simulink model "updated_simulation (2)"  (R2026b)
settings: Solver=VariableStepAuto  StopTime=15
libraries: simulink x1
settings Model: Creator=Siddhi  LastModifiedBy=Siddhi

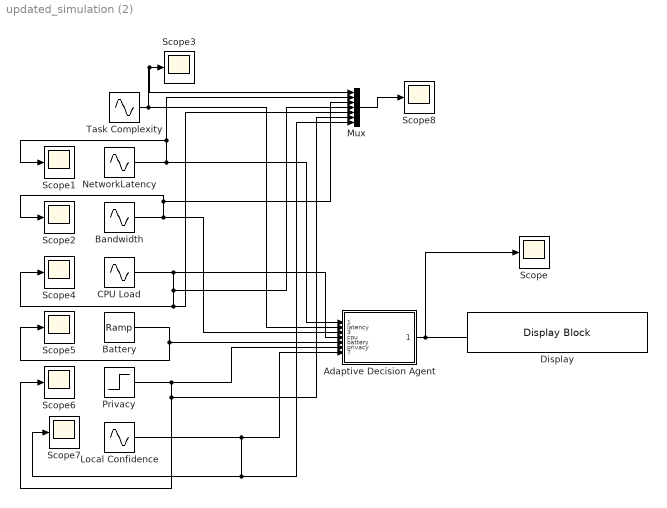
== system updated_simulation (2) ==
  Adaptive Decision Agent : MATLAB Function  TreatAsAtomicUnit=on
  Bandwidth : Sin  Amplitude=4  Bias=10  Frequency=0.12  SampleTime=0
  Battery : simulink/Sources/Ramp  slope=-0.5  start=0  InitialOutput=80
  CPU Load : Sin  Amplitude=25  Bias=60  Frequency=0.20  SampleTime=0
  Display : DisplayBlock  LabelPosition=Hide  Transparency=1  GridColor=[0.502, 0.502, 0.502]
  Local Confidence : Sin  Amplitude=0.225  Bias=0.725  Frequency=0.10  SampleTime=0
  Mux : Mux  Inputs=7
  NetworkLatency : Sin  Amplitude=20  Bias=50  Frequency=0.15  SampleTime=0
  Privacy : Step  Time=10  SampleTime=0
  Scope{,1..8} (9 alike) : Scope
      Scope settings: ActiveDisplayYMinimum=-2.4852916893203165  ActiveDisplayYMaximum=5.9778459726138227
      Scope2 settings: DataLoggingVariableName=ScopeData2
      Scope3 settings: ActiveDisplayYMinimum=0.4579264507596052  ActiveDisplayYMaximum=0.8786619431635535  DataLoggingVariableName=ScopeData3
      Scope4 settings: DataLoggingVariableName=ScopeData4
      Scope5 settings: DataLoggingVariableName=ScopeData5
      Scope6 settings: DataLoggingVariableName=ScopeData6
      Scope7 settings: DataLoggingVariableName=ScopeData7
      Scope8 settings: ActiveDisplayYMinimum=-10.624817875718643  ActiveDisplayYMaximum=95.6233608814678  DataLoggingVariableName=ScopeData8
  Task Complexity : Sin  Amplitude=0.4  Bias=0.5  Frequency=0.1  SampleTime=0
  wires:
  Task Complexity/1 -> Mux/1, Scope3/1, Adaptive Decision Agent/2(latency)
  NetworkLatency/1 -> Mux/2, Scope1/1, Adaptive Decision Agent/1(complexity)
  Adaptive Decision Agent/1(decision) -> Scope/1
  Bandwidth/1 -> Mux/3, Scope2/1, Adaptive Decision Agent/3(bandwidth)
  CPU Load/1 -> Mux/4, Scope4/1, Mux/5, Adaptive Decision Agent/4(cpu)
  Battery/1 -> Scope5/1, Adaptive Decision Agent/5(battery)
  Privacy/1 -> Mux/6, Scope6/1, Adaptive Decision Agent/6(privacy)
  Local Confidence/1 -> Scope7/1, Mux/7, Adaptive Decision Agent/7(confidence)
  Mux/1 -> Scope8/1

== matlab function updated_simulation (2)/Adaptive Decision Agent ==
  data: complexity input; decision output; latency input; bandwidth input; cpu input; battery input; privacy input; confidence input

function decision = AdaptiveDecisionAgent( ...
    complexity, latency, bandwidth, cpu, ...
    battery, privacy, confidence)

% Decision codes:
% 1 = Edge
% 2 = Cloud
% 3 = Hybrid

if privacy > 0.7
    decision = 1;

elseif latency > 60
    decision = 1;

elseif battery < 30 && cpu > 70
    decision = 2;

elseif complexity > 0.7 && ...
        bandwidth > 10 && confidence > 0.6
    decision = 2;

else
    decision = 3;
end

end
